simulink model "Template_v5_0_0_2026a_Original"  (R2026a)
settings: Solver=ode4  StopTime=tsim  FixedStep=baseRate  RelTol=1e-6  AbsTol=1e-6
undefined symbols (not defined in the file or in its folder): baseRate, dataRate, DiscIntNeverNeededParam, F_thrusters_BLACK, F_thrusters_BLUE, F_thrusters_RED, home_states_BLACK, home_states_BLUE, home_states_RED, IBLACK, IBLUE, init_states_BLACK, init_states_BLUE, init_states_RED, IRED, K_BLACK, K_BLUE, K_RED, labConsoleIP, mBLACK, mBLUE, mRED, Phase0_End, Phase1_End, Phase2_End, Phase3_End, Phase3_SubPhase1_End, Phase3_SubPhase2_End, Phase3_SubPhase3_End, Phase3_SubPhase4_End, Phase4_End, Phase5_End, platformSelection, PWMFreq, serverRate, simMode, tableDamping_BLACK, tableDamping_BLUE, tableDamping_RED, tableSlope, thrust_decay_BLACK, thrust_decay_BLUE, thrust_decay_RED, thruster_dist2CG_BLACK, thruster_dist2CG_BLUE, thruster_dist2CG_RED, xLength, yLength
libraries: simulink x18, dspinverses x3, nvidiaCommlib x1
(part 4 of 7)

== system Template_v5_0_0_2026a_Original/PhaseSpace Camera Code/Use Hardware to Obtain States/Store RED Data ==
  note: Store RED Position and Velocity Data
  RED Data : Inport
  RED Velocities : Inport  Port=2
  PS Clock : Inport  Port=3
  Calculate True Time Step : Subsystem
      settings: PortSchema="{\"entries\":[{\"content\":{\"sides\":[{\"content\":{\"connectorIds\":[\"In1\"]},\"type\":\"ConnectorPlacement.EquallySpacedRectSide\",\"uuid\":\"62932c5c-f2a7-44c8-96b4-4a75bab3a126\"},{\"content\":{\"connectorIds\":[\"Out1\"],\"side\":\"RIGHT\"},\"type\":\"ConnectorPlacement.EquallySpacedRectSide\",\"uuid\":\"82b3b717-2171-4047-b0df-3cd41cf9dfc7\"},{\"content\":{\"side\":\"TOP\"},\"type\":\"ConnectorPlacement.EquallySpacedRectSide\",\"uuid\":\"a142272a-a0ff-4882-8a2d-4633b3c7e02f\"},{\"content\":{\"connectorIds\":[\"In2\"],\"side\":\"BOTTOM\"},\"type\":\"ConnectorPlacement.EquallySpacedRectSide\",\"uuid\":\"b1e1ff4c-66d6-488f-92fb-77f76780833b\"}]},\"type\":\"ConnectorPlacement.EquallySpacedConnector\",\"uuid\":\"98c51868-8a10-4b52-aae4-56f6042c65c4\"}],\"packageUris\":[\"http://schema.mathworks.com/mf0/Connector/R2020b\"],\"version\":\"1.0\"}"
  Convert REDVX from [mm] to [m] : Gain  Gain=1/1000
  Convert REDVY from [mm] to [m] : Gain  Gain=1/1000
  Convert REDX from [mm] to [m] : Gain  Gain=1/1000
  Convert REDY from [mm] to [m] : Gain  Gain=1/1000
  Demux : Demux  Outputs=3
  Demux1 : Demux
  Demux2 : Demux  Outputs=3
  Mux{1..4} (4 alike) : Mux  Inputs=3
  RED_Px7 : DataStoreWrite  DataStoreName=RED_Measured_States  IndexOptions=Index vector (dialog)  Indices=1  OutputSizes=1
  Reshape : Reshape  OutputDimensionality=Column vector (2-D)
  Subsystem1 : Subsystem
  Subsystem2 : Subsystem
  Universal_Time : DataStoreWrite  DataStoreName=Univ_Time  IndexOptions=Index vector (dialog)  Indices=1  OutputSizes=1
  Wrap : Subsystem
  wires:
  Demux1/2 -> Convert REDX from [mm] to [m]/1
  Demux1/3 -> Convert REDY from [mm] to [m]/1
  RED Data/1 -> Demux1/1
  Demux1/4 -> Mux3/3
  Demux1/1 -> Universal_Time/1
  Mux2/1 -> RED_Px7/1
  Reshape/1 -> Subsystem1/2(y)
  Wrap/1(Wrapped Angle) -> Mux1/3
  Demux/3 -> Wrap/1(Unwrapped Angle)
  Demux/1 -> Mux1/1
  Subsystem2/1(dy/dt) -> Reshape/1
  Mux3/1 -> Subsystem2/2(y), Demux/1, Calculate True Time Step/2(Data)
  Demux/2 -> Mux1/2
  Convert REDX from [mm] to [m]/1 -> Mux3/1
  Convert REDY from [mm] to [m]/1 -> Mux3/2
  Calculate True Time Step/1(dt_out) -> Subsystem2/1(dt), Subsystem1/1(dt)
  Mux1/1 -> Mux2/1
  Subsystem1/1(dy/dt) -> Mux2/3
  Convert REDVX from [mm] to [m]/1 -> Mux4/1
  Convert REDVY from [mm] to [m]/1 -> Mux4/2
  Demux2/1 -> Convert REDVX from [mm] to [m]/1
  Demux2/2 -> Convert REDVY from [mm] to [m]/1
  Demux2/3 -> Mux4/3
  RED Velocities/1 -> Demux2/1
  Mux4/1 -> Mux2/2
  PS Clock/1 -> Calculate True Time Step/1(Time)

== system Template_v5_0_0_2026a_Original/Simulate Plant Dynamics/BLACK Dynamics/Calculated & Store Measured States ==
  y : Inport
  dt : Inport  Port=2
  Demux : Demux  Outputs=3
  Measured States for BLACK : DataStoreWrite  DataStoreName=BLACK_Measured_States  IndexOptions=Index vector (dialog)  Indices=1  OutputSizes=1
  Mux1 : Mux  Inputs=3
  Mux2 : Mux  Inputs=3
  Reshape : Reshape  OutputDimensionality=Column vector (2-D)
  Subsystem1 : Subsystem
  Subsystem2 : Subsystem
  Wrap : Subsystem
  wires:
  Demux/1 -> Mux1/1
  Wrap/1(Wrapped Angle) -> Mux1/3
  Demux/3 -> Wrap/1(Unwrapped Angle)
  Demux/2 -> Mux1/2
  Mux2/1 -> Measured States for BLACK/1
  Reshape/1 -> Subsystem1/2(y)
  Subsystem2/1(dy/dt) -> Mux2/2, Reshape/1
  y/1 -> Subsystem2/2(y), Demux/1
  Mux1/1 -> Mux2/1
  Subsystem1/1(dy/dt) -> Mux2/3
  dt/1 -> Subsystem1/1(dt), Subsystem2/1(dt)

== system Template_v5_0_0_2026a_Original/Simulate Plant Dynamics/BLACK Dynamics/Calculated & Store True States ==
  y : Inport
  Demux : Demux  Outputs=3
  Discrete Derivative : simulink/Discrete/Discrete Derivative  gainval=1.0  ICPrevScaledInput=0.0  OutMin=[]  OutMax=[]  OutDataType=fixdt(1, 16)  OutScaling=2^-10  DoSatur=off
  Discrete Derivative1 : simulink/Discrete/Discrete Derivative  gainval=1.0  ICPrevScaledInput=0.0  OutMin=[]  OutMax=[]  OutDataType=fixdt(1, 16)  OutScaling=2^-10  DoSatur=off
  Mux1 : Mux  Inputs=3
  Mux2 : Mux  Inputs=3
  True States for BLACK : DataStoreWrite  DataStoreName=BLACK_True_States  IndexOptions=Index vector (dialog)  Indices=1  OutputSizes=1
  Wrap : Subsystem
  wires:
  Demux/1 -> Mux1/1
  Wrap/1(Wrapped Angle) -> Mux1/3
  Demux/3 -> Wrap/1(Unwrapped Angle)
  Demux/2 -> Mux1/2
  Mux2/1 -> True States for BLACK/1
  y/1 -> Discrete Derivative/1, Demux/1
  Discrete Derivative/1 -> Mux2/2, Discrete Derivative1/1
  Mux1/1 -> Mux2/1
  Discrete Derivative1/1 -> Mux2/3

== system Template_v5_0_0_2026a_Original/Simulate Plant Dynamics/BLACK Dynamics/Data @ Measurement Rate ==
  Data Input : Inport
  Calculate True Time Step : Subsystem
  Constant1 : Constant  Value=dataRate
  Constant2 : Constant  Value=0
  Data Store Read : DataStoreRead  DataStoreName=Univ_Time  IndexOptions=Index vector (dialog)  Indices=1  OutputSizes=1
  Delay : Delay  DelayLength=1
  Enabled Subsystem : Subsystem  TreatAsAtomicUnit=on
  Enabled Subsystem1 : Subsystem  TreatAsAtomicUnit=on
  Relational Operator1 : RelationalOperator  OutDataTypeStr=boolean  RndMeth=Simplest  InputSameDT=off
  Relational Operator2 : RelationalOperator  Operator===  OutDataTypeStr=boolean  RndMeth=Simplest  InputSameDT=off
  Subtract : Sum  Inputs=+-
  Data Held : Outport
  Time Step : Outport  Port=2
  wires:
  Data Input/1 -> Enabled Subsystem1/1(ThrustPer_Final)
  Subtract/1 -> Relational Operator2/1, Delay/1
  Relational Operator2/1 -> Enabled Subsystem1/Enable
  Relational Operator1/1 -> Enabled Subsystem/Enable
  Constant1/1 -> Calculate True Time Step/3(Rate), Relational Operator1/2
  Constant2/1 -> Relational Operator2/2
  Enabled Subsystem/1(Out1) -> Calculate True Time Step/2(Time), Subtract/2
  Delay/1 -> Relational Operator1/1
  Data Store Read/1 -> Enabled Subsystem/1(In1), Subtract/1
  Enabled Subsystem1/1(Out1) -> Calculate True Time Step/1(Data), Data Held/1
  Calculate True Time Step/1(dt_out) -> Time Step/1

== system Template_v5_0_0_2026a_Original/Simulate Plant Dynamics/BLACK Dynamics/Dynamics Model for BLACK ==
  control_inputs : Inport
  Acceleration to Velocity : DiscreteIntegrator  IntegratorMethod=Integration: Backward Euler  SampleTime=-1  ICPrevOutput=DiscIntNeverNeededParam  ICPrevScaledInput=DiscIntNeverNeededParam
  Float State : DataStoreRead  DataStoreName=Float_State  IndexOptions=Index vector (dialog)  Indices=1  OutputSizes=1
  MATLAB Function : MATLAB Function  TreatAsAtomicUnit=on
  Previous Position : UnitDelay  InitialCondition=init_states_BLACK(:)  SampleTime=-1
  Previous Velocity : UnitDelay  InitialCondition=[0; 0; 0]  SampleTime=-1
  Velocity to Position : DiscreteIntegrator  IntegratorMethod=Integration: Backward Euler  InitialCondition=init_states_BLACK  SampleTime=-1  ICPrevOutput=DiscIntNeverNeededParam  ICPrevScaledInput=DiscIntNeverNeededParam
  states : Outport  VectorParamsAs1DForOutWhenUnconnected=off
  wires:
  control_inputs/1 -> MATLAB Function/1(control_inputs)
  MATLAB Function/1(x_ddot) -> Acceleration to Velocity/1
  Acceleration to Velocity/1 -> Velocity to Position/1, Previous Velocity/1
  Velocity to Position/1 -> states/1, Previous Position/1
  Previous Position/1 -> MATLAB Function/2(position)
  Previous Velocity/1 -> MATLAB Function/3(velocity)
  Float State/1 -> MATLAB Function/4(floating)

== system Template_v5_0_0_2026a_Original/Simulate Plant Dynamics/BLUE Dynamics/BLUE  Dynamics Model ==
  control_inputs : Inport
  Acceleration to Velocity : DiscreteIntegrator  IntegratorMethod=Integration: Backward Euler  SampleTime=-1  ICPrevOutput=DiscIntNeverNeededParam  ICPrevScaledInput=DiscIntNeverNeededParam
  Float State : DataStoreRead  DataStoreName=Float_State  IndexOptions=Index vector (dialog)  Indices=1  OutputSizes=1
  MATLAB Function : MATLAB Function  TreatAsAtomicUnit=on
  Previous Position : UnitDelay  InitialCondition=init_states_BLUE(:)  SampleTime=-1
  Previous Velocity : UnitDelay  InitialCondition=[0; 0; 0]  SampleTime=-1
  Velocity to Position : DiscreteIntegrator  IntegratorMethod=Integration: Backward Euler  InitialCondition=init_states_BLUE  SampleTime=-1  ICPrevOutput=DiscIntNeverNeededParam  ICPrevScaledInput=DiscIntNeverNeededParam
  states : Outport  VectorParamsAs1DForOutWhenUnconnected=off
  wires:
  control_inputs/1 -> MATLAB Function/1(control_inputs)
  MATLAB Function/1(x_ddot) -> Acceleration to Velocity/1
  Acceleration to Velocity/1 -> Velocity to Position/1, Previous Velocity/1
  Velocity to Position/1 -> states/1, Previous Position/1
  Previous Position/1 -> MATLAB Function/2(position)
  Previous Velocity/1 -> MATLAB Function/3(velocity)
  Float State/1 -> MATLAB Function/4(floating)

== system Template_v5_0_0_2026a_Original/Simulate Plant Dynamics/BLUE Dynamics/Calculated & Store Measured States ==
  y : Inport
  dt : Inport  Port=2
  Demux : Demux  Outputs=3
  Measured States for BLUE : DataStoreWrite  DataStoreName=BLUE_Measured_States  IndexOptions=Index vector (dialog)  Indices=1  OutputSizes=1
  Mux1 : Mux  Inputs=3
  Mux2 : Mux  Inputs=3
  Reshape : Reshape  OutputDimensionality=Column vector (2-D)
  Subsystem1 : Subsystem
  Subsystem2 : Subsystem
  Wrap : Subsystem
  wires:
  Demux/1 -> Mux1/1
  Wrap/1(Wrapped Angle) -> Mux1/3
  Demux/3 -> Wrap/1(Unwrapped Angle)
  Demux/2 -> Mux1/2
  Mux2/1 -> Measured States for BLUE/1
  Reshape/1 -> Subsystem1/2(y)
  Subsystem2/1(dy/dt) -> Mux2/2, Reshape/1
  y/1 -> Subsystem2/2(y), Demux/1
  dt/1 -> Subsystem1/1(dt), Subsystem2/1(dt)
  Subsystem1/1(dy/dt) -> Mux2/3
  Mux1/1 -> Mux2/1

== system Template_v5_0_0_2026a_Original/Simulate Plant Dynamics/BLUE Dynamics/Calculated & Store True States ==
  y : Inport
  Demux : Demux  Outputs=3
  Discrete Derivative : simulink/Discrete/Discrete Derivative  gainval=1.0  ICPrevScaledInput=0.0  OutMin=[]  OutMax=[]  OutDataType=fixdt(1, 16)  OutScaling=2^-10  DoSatur=off
  Discrete Derivative1 : simulink/Discrete/Discrete Derivative  gainval=1.0  ICPrevScaledInput=0.0  OutMin=[]  OutMax=[]  OutDataType=fixdt(1, 16)  OutScaling=2^-10  DoSatur=off
  Mux1 : Mux  Inputs=3
  Mux2 : Mux  Inputs=3
  True States for BLUE : DataStoreWrite  DataStoreName=BLUE_True_States  IndexOptions=Index vector (dialog)  Indices=1  OutputSizes=1
  Wrap : Subsystem
  wires:
  Demux/1 -> Mux1/1
  Wrap/1(Wrapped Angle) -> Mux1/3
  Demux/3 -> Wrap/1(Unwrapped Angle)
  Demux/2 -> Mux1/2
  Mux2/1 -> True States for BLUE/1
  Mux1/1 -> Mux2/1
  y/1 -> Discrete Derivative/1, Demux/1
  Discrete Derivative/1 -> Discrete Derivative1/1, Mux2/2
  Discrete Derivative1/1 -> Mux2/3

== system Template_v5_0_0_2026a_Original/Simulate Plant Dynamics/BLUE Dynamics/Data @ Measurement Rate ==
  Data Input : Inport
  Calculate True Time Step : Subsystem
  Constant1 : Constant  Value=dataRate
  Constant2 : Constant  Value=0
  Data Store Read : DataStoreRead  DataStoreName=Univ_Time  IndexOptions=Index vector (dialog)  Indices=1  OutputSizes=1
  Delay : Delay  DelayLength=1
  Enabled Subsystem : Subsystem  TreatAsAtomicUnit=on
  Enabled Subsystem1 : Subsystem  TreatAsAtomicUnit=on
  Relational Operator1 : RelationalOperator  OutDataTypeStr=boolean  RndMeth=Simplest  InputSameDT=off
  Relational Operator2 : RelationalOperator  Operator===  OutDataTypeStr=boolean  RndMeth=Simplest  InputSameDT=off
  Subtract : Sum  Inputs=+-
  Data Held : Outport
  Time Step : Outport  Port=2
  wires:
  Data Input/1 -> Enabled Subsystem1/1(ThrustPer_Final)
  Subtract/1 -> Relational Operator2/1, Delay/1
  Relational Operator2/1 -> Enabled Subsystem1/Enable
  Relational Operator1/1 -> Enabled Subsystem/Enable
  Constant1/1 -> Calculate True Time Step/3(Rate), Relational Operator1/2
  Constant2/1 -> Relational Operator2/2
  Enabled Subsystem/1(Out1) -> Calculate True Time Step/2(Time), Subtract/2
  Delay/1 -> Relational Operator1/1
  Data Store Read/1 -> Enabled Subsystem/1(In1), Subtract/1
  Enabled Subsystem1/1(Out1) -> Calculate True Time Step/1(Data), Data Held/1
  Calculate True Time Step/1(dt_out) -> Time Step/1

== system Template_v5_0_0_2026a_Original/Simulate Plant Dynamics/RED and ARM Dynamics/RED + ARM ==
  note: RED + ARM Plant (spot.arm.Plant): the base, the arm and its three Dynamixel servos in PWM control, with their back-EMF and friction, integrated at armModel.innerStep (1 ms) within each diagram step. Its arm input is what the real servos get: ARM_Controls, each joint's PWM [885 = 100 %]; it writes ARM_Measured_PWM, the PWM each servo applies. Parameters: armModel (spot.arm.parameters; friction and back-EMF from the project's arm calibration when there is one).
  Action Port : ActionPort  ActionPortLabel=if(u1 == 4 | u1 == 5 | u1 == 10 | u1 == 11)
  Add Noise : RandomNumber  Variance=1e-9  SampleTime=baseRate
  Calculated & Store Measured States : Subsystem
  Calculated & Store True States : Subsystem
  Data @ Measurement Rate : Subsystem
  Data Store Read3 : DataStoreRead  DataStoreName=ARM_Controls  IndexOptions=Index vector (dialog)  Indices=1  OutputSizes=1
  Data Store Write : DataStoreWrite  DataStoreName=ARM_Measured_States  IndexOptions=Index vector (dialog)  Indices=1  OutputSizes=1
  Data Store Write1 : DataStoreWrite  DataStoreName=ARM_Measured_PWM  IndexOptions=Index vector (dialog)  Indices=1  OutputSizes=1
  Demux : Demux  Outputs=[1,1,10]
  Encoder Pulses : Quantizer  QuantizationInterval=2*pi/4096
  Exceeded Table Limits : Subsystem
  Float State : DataStoreRead  DataStoreName=Float_State  IndexOptions=Index vector (dialog)  Indices=1  OutputSizes=1
  Joint Angles : Selector  InputPortWidth=6  IndexOptions=Index vector (dialog)  Indices=[4 5 6]  OutputSizes=1
  Joint Rates : Selector  InputPortWidth=6  IndexOptions=Index vector (dialog)  Indices=[4 5 6]  OutputSizes=1
  Mux : Mux  Inputs=2
  Mux Encoders : Mux  Inputs=2
  RED + ARM Plant : MATLABSystem  System=spot.arm.Plant  Model=armModel  FixedBase=off  FloatInput=on  SimulateUsing=Code generation
      mask Type: spot.arm.Plant
  Saturated Control Commands for RED : DataStoreRead  DataStoreName=RED_Saturated_Controls  IndexOptions=Index vector (dialog)  Indices=1  OutputSizes=1
  Stop Simulation : Stop
  Sum : Sum  Inputs=++|
  Terminator : Terminator
  Velocity Units : Quantizer  QuantizationInterval=0.229*2*pi/60
  wires:
  Data @ Measurement Rate/2(Time Step) -> Calculated & Store Measured States/2(dt)
  Mux/1 -> Demux/1
  Demux/1 -> Exceeded Table Limits/1(X)
  Exceeded Table Limits/1(Stop) -> Stop Simulation/1
  Demux/2 -> Exceeded Table Limits/2(Y)
  Demux/3 -> Terminator/1
  Add Noise/1 -> Sum/1
  Sum/1 -> Data @ Measurement Rate/1(Data Input)
  Data @ Measurement Rate/1(Data Held) -> Calculated & Store Measured States/1(y)
  Saturated Control Commands for RED/1 -> RED + ARM Plant/1
  RED + ARM Plant/1 -> Calculated & Store True States/1(y), Sum/2, Mux/1, Joint Angles/1
  RED + ARM Plant/2 -> Mux/2, Joint Rates/1
  Data Store Read3/1 -> RED + ARM Plant/2
  Joint Angles/1 -> Encoder Pulses/1
  Joint Rates/1 -> Velocity Units/1
  Encoder Pulses/1 -> Mux Encoders/1
  Velocity Units/1 -> Mux Encoders/2
  Mux Encoders/1 -> Data Store Write/1
  RED + ARM Plant/3 -> Data Store Write1/1
  Float State/1 -> RED + ARM Plant/3

== system Template_v5_0_0_2026a_Original/Simulate Plant Dynamics/RED and ARM Dynamics/RED Only ==
  Action Port : ActionPort  ActionPortLabel=else
  Add Noise : RandomNumber  Variance=1e-9  SampleTime=baseRate
  Calculated & Store Measured States : Subsystem
  Calculated & Store True States : Subsystem
  Data @ Measurement Rate : Subsystem
  Dynamics Model for RED : Subsystem  SystemSampleTime=serverRate
      settings: PortSchema="{\"entries\":[{\"content\":{\"sides\":[{\"content\":{\"connectorIds\":[\"In1\"]},\"type\":\"ConnectorPlacement.EquallySpacedRectSide\",\"uuid\":\"36f8472d-4371-4b5e-bb25-792dc7798e2d\"},{\"content\":{\"side\":\"RIGHT\"},\"type\":\"ConnectorPlacement.EquallySpacedRectSide\",\"uuid\":\"cd500640-3349-40a3-88e5-d39ca64affda\"},{\"content\":{\"connectorIds\":[\"Out1\"],\"side\":\"TOP\"},\"type\":\"ConnectorPlacement.EquallySpacedRectSide\",\"uuid\":\"f35070a8-6b00-4762-8673-30fcbcb2fe63\"}]},\"type\":\"ConnectorPlacement.EquallySpacedConnector\",\"uuid\":\"7478ab5e-be27-4ef2-a158-875ec93c8619\"}],\"packageUris\":[\"http://schema.mathworks.com/mf0/Connector/R2020b\"],\"version\":\"1.0\"}"
  Saturated Control Commands for RED : DataStoreRead  DataStoreName=RED_Saturated_Controls  IndexOptions=Index vector (dialog)  Indices=1  OutputSizes=1
  Sum : Sum  Inputs=++|
  wires:
  Saturated Control Commands for RED/1 -> Dynamics Model for RED/1(control_inputs)
  Data @ Measurement Rate/2(Time Step) -> Calculated & Store Measured States/2(dt)
  Data @ Measurement Rate/1(Data Held) -> Calculated & Store Measured States/1(y)
  Add Noise/1 -> Sum/1
  Dynamics Model for RED/1(states) -> Sum/2, Calculated & Store True States/1(y)
  Sum/1 -> Data @ Measurement Rate/1(Data Input)

== system Template_v5_0_0_2026a_Original/Thruster & Float Control Code/Change BLACK Behavior/Calculate Duty Cycle ==
  "[Fx_b; Fy_b; Tz]" : Inport
  Measured Attitude : Inport  Port=2
  Demux : Demux  Outputs=3
  Duty Cycle @ PWM : Subsystem
  Generate Initial Guess : Subsystem
  MATLAB Function1 : MATLAB Function  TreatAsAtomicUnit=on
  MATLAB Function5 : MATLAB Function  TreatAsAtomicUnit=on  mask{max_iters=20, tol=1e-6}
      mask prompts: max_iters "Maximum Number of Iterations"; tol "Convergence Tolerance"
  Mux : Mux  Inputs=2
  Mux1 : Mux  Inputs=2
  Product1 : Product  Multiplication=Matrix(*)
  Reshape : Reshape  OutputDimensionality=Column vector (2-D)
  Rotate Forces to Inertial : Subsystem
  Duty Cycle : Outport  VectorParamsAs1DForOutWhenUnconnected=off
  Saturated Forces Moments : Outport  Port=2
  wires:
  Rotate Forces to Inertial/1(F_I) -> Mux1/1
  Generate Initial Guess/1(Duty Cycle) -> MATLAB Function5/2(x0)
  Product1/1 -> Demux/1
  Measured Attitude/1 -> Rotate Forces to Inertial/2(Rz)
  Duty Cycle @ PWM/1(Duty Cycle Held) -> Product1/2
  "[Fx_b; Fy_b; Tz]"/1 -> Generate Initial Guess/1("[Fx; Fy; Tz]"), Reshape/1
  MATLAB Function5/2(duty_cycles) -> MATLAB Function1/1(ThrustPer), Duty Cycle/1
  Demux/2 -> Mux/2
  Mux/1 -> Rotate Forces to Inertial/1("F_b ")
  Demux/3 -> Mux1/2
  Demux/1 -> Mux/1
  Reshape/1 -> MATLAB Function5/1(u_desired)
  MATLAB Function5/1(H_final) -> Product1/1
  Mux1/1 -> Saturated Forces Moments/1
  MATLAB Function1/1(ThrustPer_Final) -> Duty Cycle @ PWM/1(ThrustPer_Final)

== system Template_v5_0_0_2026a_Original/Thruster & Float Control Code/Change BLACK Behavior/Rotate Forces to Body ==
  "F_I " : Inport
  Rz : Inport  Port=2
  Create Rotation Matrix : MATLAB Function  TreatAsAtomicUnit=on
  Rotate F_I to F_b : Product  Multiplication=Matrix(*)
  F_b : Outport  VectorParamsAs1DForOutWhenUnconnected=off
  wires:
  Rotate F_I to F_b/1 -> F_b/1
  Create Rotation Matrix/1(C_bI) -> Rotate F_I to F_b/1
  "F_I "/1 -> Rotate F_I to F_b/2
  Rz/1 -> Create Rotation Matrix/1(Rz)

== system Template_v5_0_0_2026a_Original/Thruster & Float Control Code/Change BLUE Behavior/Calculate Duty Cycle ==
  "[Fx_b; Fy_b; Tz]" : Inport
  Measured Attitude : Inport  Port=2
  Demux : Demux  Outputs=3
  Duty Cycle @ PWM : Subsystem
  Generate Initial Guess : Subsystem
  MATLAB Function1 : MATLAB Function  TreatAsAtomicUnit=on
  MATLAB Function5 : MATLAB Function  TreatAsAtomicUnit=on  mask{max_iters=20, tol=1e-6}
      mask prompts: max_iters "Maximum Number of Iterations"; tol "Convergence Tolerance"
  Mux : Mux  Inputs=2
  Mux1 : Mux  Inputs=2
  Product1 : Product  Multiplication=Matrix(*)
  Reshape : Reshape  OutputDimensionality=Column vector (2-D)
  Rotate Forces to Inertial : Subsystem
  Duty Cycle : Outport  VectorParamsAs1DForOutWhenUnconnected=off
  Saturated Forces Moments : Outport  Port=2
  wires:
  Rotate Forces to Inertial/1(F_I) -> Mux1/1
  Generate Initial Guess/1(Duty Cycle) -> MATLAB Function5/2(x0)
  Product1/1 -> Demux/1
  Measured Attitude/1 -> Rotate Forces to Inertial/2(Rz)
  Duty Cycle @ PWM/1(Duty Cycle Held) -> Product1/2
  "[Fx_b; Fy_b; Tz]"/1 -> Generate Initial Guess/1("[Fx; Fy; Tz]"), Reshape/1
  MATLAB Function5/2(duty_cycles) -> Duty Cycle/1, MATLAB Function1/1(ThrustPer)
  Demux/2 -> Mux/2
  Mux/1 -> Rotate Forces to Inertial/1("F_b ")
  Demux/3 -> Mux1/2
  Demux/1 -> Mux/1
  Reshape/1 -> MATLAB Function5/1(u_desired)
  Mux1/1 -> Saturated Forces Moments/1
  MATLAB Function5/1(H_final) -> Product1/1
  MATLAB Function1/1(ThrustPer_Final) -> Duty Cycle @ PWM/1(ThrustPer_Final)

== system Template_v5_0_0_2026a_Original/Thruster & Float Control Code/Change BLUE Behavior/Rotate Forces to Body ==
  "F_I " : Inport
  Rz : Inport  Port=2
  Create Rotation Matrix : MATLAB Function  TreatAsAtomicUnit=on
  Rotate F_I to F_b : Product  Multiplication=Matrix(*)
  F_b : Outport  VectorParamsAs1DForOutWhenUnconnected=off
  wires:
  Rotate F_I to F_b/1 -> F_b/1
  Create Rotation Matrix/1(C_bI) -> Rotate F_I to F_b/1
  "F_I "/1 -> Rotate F_I to F_b/2
  Rz/1 -> Create Rotation Matrix/1(Rz)

== system Template_v5_0_0_2026a_Original/Thruster & Float Control Code/Change RED Behavior/Calculate Duty Cycle ==
  "[Fx_b; Fy_b; Tz]" : Inport
  Measured Attitude : Inport  Port=2
  Demux : Demux  Outputs=3
  Duty Cycle @ PWM : Subsystem
  Generate Initial Guess : Subsystem
  MATLAB Function5 : MATLAB Function  TreatAsAtomicUnit=on  mask{max_iters=20, tol=1e-6}
      mask prompts: max_iters "Maximum Number of Iterations"; tol "Convergence Tolerance"
  MATLAB Function8 : MATLAB Function  TreatAsAtomicUnit=on
  Mux : Mux  Inputs=2
  Mux1 : Mux  Inputs=2
  Product1 : Product  Multiplication=Matrix(*)
  Reshape : Reshape  OutputDimensionality=Column vector (2-D)
  Rotate Forces to Inertial : Subsystem
  Duty Cycle : Outport  VectorParamsAs1DForOutWhenUnconnected=off
  Saturated Forces Moments : Outport  Port=2
  wires:
  Demux/2 -> Mux/2
  Measured Attitude/1 -> Rotate Forces to Inertial/2(Rz)
  Rotate Forces to Inertial/1(F_I) -> Mux1/1
  Product1/1 -> Demux/1
  Demux/1 -> Mux/1
  Mux/1 -> Rotate Forces to Inertial/1("F_b ")
  Demux/3 -> Mux1/2
  Reshape/1 -> MATLAB Function5/1(u_desired)
  MATLAB Function5/1(H_final) -> Product1/1
  MATLAB Function5/2(duty_cycles) -> Duty Cycle/1, MATLAB Function8/1(ThrustPer)
  Duty Cycle @ PWM/1(Duty Cycle Held) -> Product1/2
  Generate Initial Guess/1(Duty Cycle) -> MATLAB Function5/2(x0)
  Mux1/1 -> Saturated Forces Moments/1
  MATLAB Function8/1(ThrustPer_Final) -> Duty Cycle @ PWM/1(ThrustPer_Final)
  "[Fx_b; Fy_b; Tz]"/1 -> Reshape/1, Generate Initial Guess/1("[Fx; Fy; Tz]")

== system Template_v5_0_0_2026a_Original/Thruster & Float Control Code/Change RED Behavior/Rotate Forces to Body ==
  "F_I " : Inport
  Rz : Inport  Port=2
  Create Rotation Matrix : MATLAB Function  TreatAsAtomicUnit=on
  Rotate F_I to F_b : Product  Multiplication=Matrix(*)
  F_b : Outport  VectorParamsAs1DForOutWhenUnconnected=off
  wires:
  Rotate F_I to F_b/1 -> F_b/1
  Create Rotation Matrix/1(C_bI) -> Rotate F_I to F_b/1
  "F_I "/1 -> Rotate F_I to F_b/2
  Rz/1 -> Create Rotation Matrix/1(Rz)

== system Template_v5_0_0_2026a_Original/1 - Experiment Logic/Phase #3: Experiment/Sub-Phase #1/Desired Joint Angles RED ==
  Constant1 : Constant  Value=pi/2
  Constant2 : Constant  Value=0
  Constant3 : Constant  Value=0
  Mux : Mux  Inputs=3
  Target Array : Outport
  wires:
  Mux/1 -> Target Array/1
  Constant3/1 -> Mux/1
  Constant1/1 -> Mux/2
  Constant2/1 -> Mux/3

== system Template_v5_0_0_2026a_Original/1 - Experiment Logic/Phase #3: Experiment/Sub-Phase #1/Desired Position BLACK ==
  Calculate Circular Tracking : Subsystem
  Calculate Time since Phase #3 Start : Subsystem
  Constant : Constant  Value=2*pi/3
  "Desired Rate " : Constant  Value=0.03490659  SampleTime=-1
  Mux : Mux  Inputs=3
  Product : Product
  Sum : Sum  Inputs=|++
  Wrap : Subsystem
  Target Array : Outport
  wires:
  Mux/1 -> Target Array/1
  Calculate Time since Phase #3 Start/1(Time) -> Product/2
  Constant/1 -> Calculate Circular Tracking/2(Phase), Sum/2
  "Desired Rate "/1 -> Product/1
  Product/1 -> Calculate Circular Tracking/1(Angular Frequency), Sum/1
  Sum/1 -> Wrap/1(In1)
  Wrap/1(Out1) -> Mux/3
  Calculate Circular Tracking/1(Target X) -> Mux/1
  Calculate Circular Tracking/2(Target Y) -> Mux/2

== system Template_v5_0_0_2026a_Original/1 - Experiment Logic/Phase #3: Experiment/Sub-Phase #1/Desired Position BLUE ==
  Calculate Circular Tracking : Subsystem
  Calculate Time since Phase #3 Start : Subsystem
  Constant : Constant  Value=4*pi/3
  "Desired Rate " : Constant  Value=0.03490659  SampleTime=-1
  Mux : Mux  Inputs=3
  Product : Product
  Sum : Sum  Inputs=|++
  Wrap : Subsystem
  Target Array : Outport
  wires:
  Mux/1 -> Target Array/1
  Calculate Time since Phase #3 Start/1(Time) -> Product/2
  Constant/1 -> Calculate Circular Tracking/2(Phase), Sum/2
  "Desired Rate "/1 -> Product/1
  Product/1 -> Calculate Circular Tracking/1(Angular Frequency), Sum/1
  Sum/1 -> Wrap/1(In1)
  Wrap/1(Out1) -> Mux/3
  Calculate Circular Tracking/1(Target X) -> Mux/1
  Calculate Circular Tracking/2(Target Y) -> Mux/2

== system Template_v5_0_0_2026a_Original/1 - Experiment Logic/Phase #3: Experiment/Sub-Phase #1/Desired Position RED ==
  Calculate Circular Tracking : Subsystem
  Calculate Time since Phase #3 Start : Subsystem
  Constant : Constant  Value=0
  "Desired Rate " : Constant  Value=0.03490659  SampleTime=-1
  Mux : Mux  Inputs=3
  Product : Product
  Sum : Sum  Inputs=|++
  Wrap : Subsystem
  Target Array : Outport
  wires:
  Mux/1 -> Target Array/1
  Calculate Time since Phase #3 Start/1(Time) -> Product/2
  Constant/1 -> Calculate Circular Tracking/2(Phase), Sum/2
  "Desired Rate "/1 -> Product/1
  Product/1 -> Calculate Circular Tracking/1(Angular Frequency), Sum/1
  Sum/1 -> Wrap/1(In1)
  Wrap/1(Out1) -> Mux/3
  Calculate Circular Tracking/1(Target X) -> Mux/1
  Calculate Circular Tracking/2(Target Y) -> Mux/2

== system Template_v5_0_0_2026a_Original/1 - Experiment Logic/Phase #3: Experiment/Sub-Phase #2/Desired Joint Angles RED ==
  Constant1 : Constant  Value=pi/2
  Constant2 : Constant  Value=0
  Constant3 : Constant  Value=pi/2
  Mux : Mux  Inputs=3
  Target Array : Outport
  wires:
  Mux/1 -> Target Array/1
  Constant3/1 -> Mux/1
  Constant1/1 -> Mux/2
  Constant2/1 -> Mux/3

== system Template_v5_0_0_2026a_Original/1 - Experiment Logic/Phase #3: Experiment/Sub-Phase #2/Desired Position BLACK ==
  Calculate Circular Tracking : Subsystem
  Calculate Time since Phase #3 Start : Subsystem
  Constant : Constant  Value=2*pi/3
  "Desired Rate " : Constant  Value=0.03490659  SampleTime=-1
  Mux : Mux  Inputs=3
  Product : Product
  Sum : Sum  Inputs=|++
  Wrap : Subsystem
  Target Array : Outport
  wires:
  Mux/1 -> Target Array/1
  Calculate Time since Phase #3 Start/1(Time) -> Product/2
  Constant/1 -> Calculate Circular Tracking/2(Phase), Sum/2
  "Desired Rate "/1 -> Product/1
  Product/1 -> Calculate Circular Tracking/1(Angular Frequency), Sum/1
  Sum/1 -> Wrap/1(In1)
  Wrap/1(Out1) -> Mux/3
  Calculate Circular Tracking/1(Target X) -> Mux/1
  Calculate Circular Tracking/2(Target Y) -> Mux/2

== system Template_v5_0_0_2026a_Original/1 - Experiment Logic/Phase #3: Experiment/Sub-Phase #2/Desired Position BLUE ==
  Calculate Circular Tracking : Subsystem
  Calculate Time since Phase #3 Start : Subsystem
  Constant : Constant  Value=4*pi/3
  "Desired Rate " : Constant  Value=0.03490659  SampleTime=-1
  Mux : Mux  Inputs=3
  Product : Product
  Sum : Sum  Inputs=|++
  Wrap : Subsystem
  Target Array : Outport
  wires:
  Mux/1 -> Target Array/1
  Calculate Time since Phase #3 Start/1(Time) -> Product/2
  Constant/1 -> Calculate Circular Tracking/2(Phase), Sum/2
  "Desired Rate "/1 -> Product/1
  Product/1 -> Calculate Circular Tracking/1(Angular Frequency), Sum/1
  Sum/1 -> Wrap/1(In1)
  Wrap/1(Out1) -> Mux/3
  Calculate Circular Tracking/1(Target X) -> Mux/1
  Calculate Circular Tracking/2(Target Y) -> Mux/2

== system Template_v5_0_0_2026a_Original/1 - Experiment Logic/Phase #3: Experiment/Sub-Phase #2/Desired Position RED ==
  Calculate Circular Tracking : Subsystem
  Calculate Time since Phase #3 Start : Subsystem
  Constant : Constant  Value=0
  "Desired Rate " : Constant  Value=0.03490659  SampleTime=-1
  Mux : Mux  Inputs=3
  Product : Product
  Sum : Sum  Inputs=|++
  Wrap : Subsystem
  Target Array : Outport
  wires:
  Mux/1 -> Target Array/1
  Calculate Time since Phase #3 Start/1(Time) -> Product/2
  Constant/1 -> Calculate Circular Tracking/2(Phase), Sum/2
  "Desired Rate "/1 -> Product/1
  Product/1 -> Calculate Circular Tracking/1(Angular Frequency), Sum/1
  Sum/1 -> Wrap/1(In1)
  Wrap/1(Out1) -> Mux/3
  Calculate Circular Tracking/1(Target X) -> Mux/1
  Calculate Circular Tracking/2(Target Y) -> Mux/2

== system Template_v5_0_0_2026a_Original/1 - Experiment Logic/Phase #3: Experiment/Sub-Phase #3/Desired Joint Angles RED ==
  Constant1 : Constant  Value=pi/2
  Constant2 : Constant  Value=0
  Constant3 : Constant  Value=pi/2
  Mux : Mux  Inputs=3
  Target Array : Outport
  wires:
  Mux/1 -> Target Array/1
  Constant3/1 -> Mux/1
  Constant1/1 -> Mux/2
  Constant2/1 -> Mux/3

== system Template_v5_0_0_2026a_Original/1 - Experiment Logic/Phase #3: Experiment/Sub-Phase #3/Desired Position BLACK ==
  Calculate Circular Tracking : Subsystem
  Calculate Time since Phase #3 Start : Subsystem
  Constant : Constant  Value=2*pi/3
  "Desired Rate " : Constant  Value=0.03490659  SampleTime=-1
  Mux : Mux  Inputs=3
  Product : Product
  Sum : Sum  Inputs=|++
  Wrap : Subsystem
  Target Array : Outport
  wires:
  Mux/1 -> Target Array/1
  Calculate Time since Phase #3 Start/1(Time) -> Product/2
  Constant/1 -> Calculate Circular Tracking/2(Phase), Sum/2
  "Desired Rate "/1 -> Product/1
  Product/1 -> Calculate Circular Tracking/1(Angular Frequency), Sum/1
  Sum/1 -> Wrap/1(In1)
  Wrap/1(Out1) -> Mux/3
  Calculate Circular Tracking/1(Target X) -> Mux/1
  Calculate Circular Tracking/2(Target Y) -> Mux/2

== system Template_v5_0_0_2026a_Original/1 - Experiment Logic/Phase #3: Experiment/Sub-Phase #3/Desired Position BLUE ==
  Calculate Circular Tracking : Subsystem
  Calculate Time since Phase #3 Start : Subsystem
  Constant : Constant  Value=4*pi/3
  "Desired Rate " : Constant  Value=0.03490659  SampleTime=-1
  Mux : Mux  Inputs=3
  Product : Product
  Sum : Sum  Inputs=|++
  Wrap : Subsystem
  Target Array : Outport
  wires:
  Mux/1 -> Target Array/1
  Calculate Time since Phase #3 Start/1(Time) -> Product/2
  Constant/1 -> Calculate Circular Tracking/2(Phase), Sum/2
  "Desired Rate "/1 -> Product/1
  Product/1 -> Calculate Circular Tracking/1(Angular Frequency), Sum/1
  Sum/1 -> Wrap/1(In1)
  Wrap/1(Out1) -> Mux/3
  Calculate Circular Tracking/1(Target X) -> Mux/1
  Calculate Circular Tracking/2(Target Y) -> Mux/2

== system Template_v5_0_0_2026a_Original/1 - Experiment Logic/Phase #3: Experiment/Sub-Phase #3/Desired Position RED ==
  Calculate Circular Tracking : Subsystem
  Calculate Time since Phase #3 Start : Subsystem
  Constant : Constant  Value=0
  "Desired Rate " : Constant  Value=0.03490659  SampleTime=-1
  Mux : Mux  Inputs=3
  Product : Product
  Sum : Sum  Inputs=|++
  Wrap : Subsystem
  Target Array : Outport
  wires:
  Mux/1 -> Target Array/1
  Calculate Time since Phase #3 Start/1(Time) -> Product/2
  Constant/1 -> Calculate Circular Tracking/2(Phase), Sum/2
  "Desired Rate "/1 -> Product/1
  Product/1 -> Calculate Circular Tracking/1(Angular Frequency), Sum/1
  Sum/1 -> Wrap/1(In1)
  Wrap/1(Out1) -> Mux/3
  Calculate Circular Tracking/1(Target X) -> Mux/1
  Calculate Circular Tracking/2(Target Y) -> Mux/2

== system Template_v5_0_0_2026a_Original/1 - Experiment Logic/Phase #3: Experiment/Sub-Phase #4/Desired Joint Angles RED ==
  Constant1 : Constant  Value=pi/2
  Constant2 : Constant  Value=0
  Constant3 : Constant  Value=pi/2
  Mux : Mux  Inputs=3
  Target Array : Outport
  wires:
  Mux/1 -> Target Array/1
  Constant3/1 -> Mux/1
  Constant1/1 -> Mux/2
  Constant2/1 -> Mux/3

== system Template_v5_0_0_2026a_Original/1 - Experiment Logic/Phase #3: Experiment/Sub-Phase #4/Desired Position BLACK ==
  Calculate Circular Tracking : Subsystem
  Calculate Time since Phase #3 Start : Subsystem
  Constant : Constant  Value=2*pi/3
  "Desired Rate " : Constant  Value=0.03490659  SampleTime=-1
  Mux : Mux  Inputs=3
  Product : Product
  Sum : Sum  Inputs=|++
  Wrap : Subsystem
  Target Array : Outport
  wires:
  Mux/1 -> Target Array/1
  Calculate Time since Phase #3 Start/1(Time) -> Product/2
  Constant/1 -> Calculate Circular Tracking/2(Phase), Sum/2
  "Desired Rate "/1 -> Product/1
  Product/1 -> Calculate Circular Tracking/1(Angular Frequency), Sum/1
  Sum/1 -> Wrap/1(In1)
  Wrap/1(Out1) -> Mux/3
  Calculate Circular Tracking/1(Target X) -> Mux/1
  Calculate Circular Tracking/2(Target Y) -> Mux/2

== system Template_v5_0_0_2026a_Original/1 - Experiment Logic/Phase #3: Experiment/Sub-Phase #4/Desired Position BLUE ==
  Calculate Circular Tracking : Subsystem
  Calculate Time since Phase #3 Start : Subsystem
  Constant : Constant  Value=4*pi/3
  "Desired Rate " : Constant  Value=0.03490659  SampleTime=-1
  Mux : Mux  Inputs=3
  Product : Product
  Sum : Sum  Inputs=|++
  Wrap : Subsystem
  Target Array : Outport
  wires:
  Mux/1 -> Target Array/1
  Calculate Time since Phase #3 Start/1(Time) -> Product/2
  Constant/1 -> Calculate Circular Tracking/2(Phase), Sum/2
  "Desired Rate "/1 -> Product/1
  Product/1 -> Calculate Circular Tracking/1(Angular Frequency), Sum/1
  Sum/1 -> Wrap/1(In1)
  Wrap/1(Out1) -> Mux/3
  Calculate Circular Tracking/1(Target X) -> Mux/1
  Calculate Circular Tracking/2(Target Y) -> Mux/2

== system Template_v5_0_0_2026a_Original/1 - Experiment Logic/Phase #3: Experiment/Sub-Phase #4/Desired Position RED ==
  Calculate Circular Tracking : Subsystem
  Calculate Time since Phase #3 Start : Subsystem
  Constant : Constant  Value=0
  "Desired Rate " : Constant  Value=0.03490659  SampleTime=-1
  Mux : Mux  Inputs=3
  Product : Product
  Sum : Sum  Inputs=|++
  Wrap : Subsystem
  Target Array : Outport
  wires:
  Mux/1 -> Target Array/1
  Calculate Time since Phase #3 Start/1(Time) -> Product/2
  Constant/1 -> Calculate Circular Tracking/2(Phase), Sum/2
  "Desired Rate "/1 -> Product/1
  Product/1 -> Calculate Circular Tracking/1(Angular Frequency), Sum/1
  Sum/1 -> Wrap/1(In1)
  Wrap/1(Out1) -> Mux/3
  Calculate Circular Tracking/1(Target X) -> Mux/1
  Calculate Circular Tracking/2(Target Y) -> Mux/2

== system Template_v5_0_0_2026a_Original/PhaseSpace Camera Code/Use Hardware to Obtain States/Receive and Process Phasespace Data/Experiment Clock ==
  packet : Inport
  age : Inport  Port=2
  Experiment Time : MATLAB Function  TreatAsAtomicUnit=on
  Send Sync. Time : Subsystem
  state : Terminator
  ClockAdjusted : Outport
  wires:
  packet/1 -> Experiment Time/1(packet)
  age/1 -> Experiment Time/2(age)
  Experiment Time/1(t) -> ClockAdjusted/1, Send Sync. Time/1(Universal Time)
  Experiment Time/2(state) -> state/1

== system Template_v5_0_0_2026a_Original/PhaseSpace Camera Code/Use Hardware to Obtain States/Store BLACK Data/Calculate True Time Step ==
  Time : Inport
  Data : Inport  Port=2
  Constant : Constant  Value=dataRate
  Constant3 : Constant  Value=0
  Delay1 : Delay  DelayLength=1  InitialCondition=0
  Delay2 : Delay  DelayLength=1  InitialCondition=0
  Demux : Demux  Outputs=3
  Enabled Subsystem3 : Subsystem  TreatAsAtomicUnit=on
  MATLAB Function : MATLAB Function  TreatAsAtomicUnit=on
  Relational Operator : RelationalOperator  Operator=~=  OutDataTypeStr=boolean  RndMeth=Simplest  InputSameDT=off
  Subtract1 : Sum  Inputs=+-
  Subtract2 : Sum  Inputs=+-
  Terminator : Terminator
  Terminator1 : Terminator
  dt_out : Outport
  wires:
  Demux/3 -> Terminator1/1
  Constant/1 -> MATLAB Function/2(dataRate)
  MATLAB Function/1(dt_out) -> dt_out/1
  Time/1 -> Delay2/1, Subtract1/1
  Enabled Subsystem3/1(dy(t)/dt) -> MATLAB Function/1(dt)
  Data/1 -> Demux/1
  Subtract2/1 -> Relational Operator/1
  Relational Operator/1 -> Enabled Subsystem3/Enable
  Constant3/1 -> Relational Operator/2
  Demux/1 -> Subtract2/1, Delay1/1
  Delay1/1 -> Subtract2/2
  Demux/2 -> Terminator/1
  Subtract1/1 -> Enabled Subsystem3/1(y2-y1)
  Delay2/1 -> Subtract1/2

== system Template_v5_0_0_2026a_Original/PhaseSpace Camera Code/Use Hardware to Obtain States/Store BLACK Data/Subsystem1 ==
  dt : Inport
  y : Inport  Port=2
  Constant3 : Constant  Value=0
  Delay1 : Delay  DelayLength=1
  Enabled Subsystem : Subsystem  TreatAsAtomicUnit=on
  Relational Operator : RelationalOperator  Operator=~=  OutDataTypeStr=boolean  RndMeth=Simplest  InputSameDT=off
  Subtract1 : Sum  Inputs=+-
  dy/dt : Outport
  wires:
  Constant3/1 -> Relational Operator/2
  Relational Operator/1 -> Enabled Subsystem/Enable
  Delay1/1 -> Subtract1/2
  dt/1 -> Enabled Subsystem/2(dt)
  Subtract1/1 -> Relational Operator/1
  Enabled Subsystem/1(dy/dt) -> dy/dt/1
  y/1 -> Enabled Subsystem/1(y), Delay1/1, Subtract1/1

== system Template_v5_0_0_2026a_Original/PhaseSpace Camera Code/Use Hardware to Obtain States/Store BLACK Data/Subsystem2 ==
  dt : Inport
  y : Inport  Port=2
  Constant3 : Constant  Value=0
  Delay1 : Delay  DelayLength=1
  Enabled Subsystem : Subsystem  TreatAsAtomicUnit=on
  Relational Operator : RelationalOperator  Operator=~=  OutDataTypeStr=boolean  RndMeth=Simplest  InputSameDT=off
  Subtract1 : Sum  Inputs=+-
  dy/dt : Outport
  wires:
  Constant3/1 -> Relational Operator/2
  Relational Operator/1 -> Enabled Subsystem/Enable
  Delay1/1 -> Subtract1/2
  dt/1 -> Enabled Subsystem/2(dt)
  Subtract1/1 -> Relational Operator/1
  Enabled Subsystem/1(dy/dt) -> dy/dt/1
  y/1 -> Enabled Subsystem/1(y), Delay1/1, Subtract1/1

== system Template_v5_0_0_2026a_Original/PhaseSpace Camera Code/Use Hardware to Obtain States/Store BLACK Data/Wrap ==
  Unwrapped Angle : Inport
  Atan2 : Trigonometry  Operator=atan2
  Cos : Trigonometry  Operator=cos
  Sin : Trigonometry
  Wrapped Angle : Outport
  wires:
  Unwrapped Angle/1 -> Sin/1, Cos/1
  Cos/1 -> Atan2/2
  Atan2/1 -> Wrapped Angle/1
  Sin/1 -> Atan2/1

== system Template_v5_0_0_2026a_Original/PhaseSpace Camera Code/Use Hardware to Obtain States/Store BLUE Data/Calculate True Time Step ==
  Time : Inport
  Data : Inport  Port=2
  Constant : Constant  Value=dataRate
  Constant3 : Constant  Value=0
  Delay1 : Delay  DelayLength=1  InitialCondition=0
  Delay2 : Delay  DelayLength=1  InitialCondition=0
  Demux : Demux  Outputs=3
  Enabled Subsystem3 : Subsystem  TreatAsAtomicUnit=on
  MATLAB Function : MATLAB Function  TreatAsAtomicUnit=on
  Relational Operator : RelationalOperator  Operator=~=  OutDataTypeStr=boolean  RndMeth=Simplest  InputSameDT=off
  Subtract1 : Sum  Inputs=+-
  Subtract2 : Sum  Inputs=+-
  Terminator : Terminator
  Terminator1 : Terminator
  dt_out : Outport
  wires:
  Demux/3 -> Terminator1/1
  Constant/1 -> MATLAB Function/2(dataRate)
  MATLAB Function/1(dt_out) -> dt_out/1
  Time/1 -> Delay2/1, Subtract1/1
  Enabled Subsystem3/1(dy(t)/dt) -> MATLAB Function/1(dt)
  Data/1 -> Demux/1
  Subtract2/1 -> Relational Operator/1
  Relational Operator/1 -> Enabled Subsystem3/Enable
  Constant3/1 -> Relational Operator/2
  Demux/1 -> Subtract2/1, Delay1/1
  Delay1/1 -> Subtract2/2
  Demux/2 -> Terminator/1
  Subtract1/1 -> Enabled Subsystem3/1(y2-y1)
  Delay2/1 -> Subtract1/2

== system Template_v5_0_0_2026a_Original/PhaseSpace Camera Code/Use Hardware to Obtain States/Store BLUE Data/Subsystem1 ==
  dt : Inport
  y : Inport  Port=2
  Constant3 : Constant  Value=0
  Delay1 : Delay  DelayLength=1
  Enabled Subsystem : Subsystem  TreatAsAtomicUnit=on
  Relational Operator : RelationalOperator  Operator=~=  OutDataTypeStr=boolean  RndMeth=Simplest  InputSameDT=off
  Subtract1 : Sum  Inputs=+-
  dy/dt : Outport
  wires:
  Constant3/1 -> Relational Operator/2
  Relational Operator/1 -> Enabled Subsystem/Enable
  Delay1/1 -> Subtract1/2
  dt/1 -> Enabled Subsystem/2(dt)
  Subtract1/1 -> Relational Operator/1
  Enabled Subsystem/1(dy/dt) -> dy/dt/1
  y/1 -> Enabled Subsystem/1(y), Delay1/1, Subtract1/1

== system Template_v5_0_0_2026a_Original/PhaseSpace Camera Code/Use Hardware to Obtain States/Store BLUE Data/Subsystem2 ==
  dt : Inport
  y : Inport  Port=2
  Constant3 : Constant  Value=0
  Delay1 : Delay  DelayLength=1
  Enabled Subsystem : Subsystem  TreatAsAtomicUnit=on
  Relational Operator : RelationalOperator  Operator=~=  OutDataTypeStr=boolean  RndMeth=Simplest  InputSameDT=off
  Subtract1 : Sum  Inputs=+-
  dy/dt : Outport
  wires:
  Constant3/1 -> Relational Operator/2
  Relational Operator/1 -> Enabled Subsystem/Enable
  Delay1/1 -> Subtract1/2
  dt/1 -> Enabled Subsystem/2(dt)
  Subtract1/1 -> Relational Operator/1
  Enabled Subsystem/1(dy/dt) -> dy/dt/1
  y/1 -> Enabled Subsystem/1(y), Delay1/1, Subtract1/1

== system Template_v5_0_0_2026a_Original/PhaseSpace Camera Code/Use Hardware to Obtain States/Store BLUE Data/Wrap ==
  Unwrapped Angle : Inport
  Atan2 : Trigonometry  Operator=atan2
  Cos : Trigonometry  Operator=cos
  Sin : Trigonometry
  Wrapped Angle : Outport
  wires:
  Unwrapped Angle/1 -> Sin/1, Cos/1
  Cos/1 -> Atan2/2
  Atan2/1 -> Wrapped Angle/1
  Sin/1 -> Atan2/1

== system Template_v5_0_0_2026a_Original/PhaseSpace Camera Code/Use Hardware to Obtain States/Store RED Data/Calculate True Time Step ==
  Time : Inport
  Data : Inport  Port=2
  Constant : Constant  Value=dataRate
  Constant3 : Constant  Value=0
  Delay1 : Delay  DelayLength=1  InitialCondition=0
  Delay2 : Delay  DelayLength=1  InitialCondition=0
  Demux : Demux  Outputs=3
  Enabled Subsystem3 : Subsystem  TreatAsAtomicUnit=on
  MATLAB Function : MATLAB Function  TreatAsAtomicUnit=on
  Relational Operator : RelationalOperator  Operator=~=  OutDataTypeStr=boolean  RndMeth=Simplest  InputSameDT=off
  Subtract1 : Sum  Inputs=+-
  Subtract2 : Sum  Inputs=+-
  Terminator : Terminator
  Terminator1 : Terminator
  dt_out : Outport
  wires:
  Demux/3 -> Terminator1/1
  Constant/1 -> MATLAB Function/2(dataRate)
  MATLAB Function/1(dt_out) -> dt_out/1
  Time/1 -> Delay2/1, Subtract1/1
  Enabled Subsystem3/1(dy(t)/dt) -> MATLAB Function/1(dt)
  Data/1 -> Demux/1
  Subtract2/1 -> Relational Operator/1
  Relational Operator/1 -> Enabled Subsystem3/Enable
  Constant3/1 -> Relational Operator/2
  Demux/1 -> Subtract2/1, Delay1/1
  Delay1/1 -> Subtract2/2
  Demux/2 -> Terminator/1
  Subtract1/1 -> Enabled Subsystem3/1(y2-y1)
  Delay2/1 -> Subtract1/2

== system Template_v5_0_0_2026a_Original/PhaseSpace Camera Code/Use Hardware to Obtain States/Store RED Data/Subsystem1 ==
  dt : Inport
  y : Inport  Port=2
  Constant3 : Constant  Value=0
  Delay1 : Delay  DelayLength=1
  Enabled Subsystem : Subsystem  TreatAsAtomicUnit=on
  Relational Operator : RelationalOperator  Operator=~=  OutDataTypeStr=boolean  RndMeth=Simplest  InputSameDT=off
  Subtract1 : Sum  Inputs=+-
  dy/dt : Outport
  wires:
  Constant3/1 -> Relational Operator/2
  Relational Operator/1 -> Enabled Subsystem/Enable
  Delay1/1 -> Subtract1/2
  dt/1 -> Enabled Subsystem/2(dt)
  Subtract1/1 -> Relational Operator/1
  Enabled Subsystem/1(dy/dt) -> dy/dt/1
  y/1 -> Enabled Subsystem/1(y), Delay1/1, Subtract1/1

== system Template_v5_0_0_2026a_Original/PhaseSpace Camera Code/Use Hardware to Obtain States/Store RED Data/Subsystem2 ==
  dt : Inport
  y : Inport  Port=2
  Constant3 : Constant  Value=0
  Delay1 : Delay  DelayLength=1
  Enabled Subsystem : Subsystem  TreatAsAtomicUnit=on
  Relational Operator : RelationalOperator  Operator=~=  OutDataTypeStr=boolean  RndMeth=Simplest  InputSameDT=off
  Subtract1 : Sum  Inputs=+-
  dy/dt : Outport
  wires:
  Constant3/1 -> Relational Operator/2
  Relational Operator/1 -> Enabled Subsystem/Enable
  Delay1/1 -> Subtract1/2
  dt/1 -> Enabled Subsystem/2(dt)
  Subtract1/1 -> Relational Operator/1
  Enabled Subsystem/1(dy/dt) -> dy/dt/1
  y/1 -> Enabled Subsystem/1(y), Delay1/1, Subtract1/1

== system Template_v5_0_0_2026a_Original/PhaseSpace Camera Code/Use Hardware to Obtain States/Store RED Data/Wrap ==
  Unwrapped Angle : Inport
  Atan2 : Trigonometry  Operator=atan2
  Cos : Trigonometry  Operator=cos
  Sin : Trigonometry
  Wrapped Angle : Outport
  wires:
  Unwrapped Angle/1 -> Sin/1, Cos/1
  Cos/1 -> Atan2/2
  Atan2/1 -> Wrapped Angle/1
  Sin/1 -> Atan2/1

== system Template_v5_0_0_2026a_Original/Simulate Plant Dynamics/BLACK Dynamics/Calculated & Store Measured States/Subsystem1 ==
  dt : Inport
  y : Inport  Port=2
  Constant3 : Constant  Value=0
  Delay1 : Delay  DelayLength=1
  Enabled Subsystem : Subsystem  TreatAsAtomicUnit=on
  Relational Operator : RelationalOperator  Operator=~=  OutDataTypeStr=boolean  RndMeth=Simplest  InputSameDT=off
  Subtract1 : Sum  Inputs=+-
  dy/dt : Outport
  wires:
  Constant3/1 -> Relational Operator/2
  Relational Operator/1 -> Enabled Subsystem/Enable
  Delay1/1 -> Subtract1/2
  dt/1 -> Enabled Subsystem/2(dt)
  Subtract1/1 -> Relational Operator/1
  Enabled Subsystem/1(dy/dt) -> dy/dt/1
  y/1 -> Enabled Subsystem/1(y), Delay1/1, Subtract1/1

== system Template_v5_0_0_2026a_Original/Simulate Plant Dynamics/BLACK Dynamics/Calculated & Store Measured States/Subsystem2 ==
  dt : Inport
  y : Inport  Port=2
  Constant3 : Constant  Value=0
  Delay1 : Delay  DelayLength=1
  Enabled Subsystem : Subsystem  TreatAsAtomicUnit=on
  Relational Operator : RelationalOperator  Operator=~=  OutDataTypeStr=boolean  RndMeth=Simplest  InputSameDT=off
  Subtract1 : Sum  Inputs=+-
  dy/dt : Outport
  wires:
  Constant3/1 -> Relational Operator/2
  Relational Operator/1 -> Enabled Subsystem/Enable
  Delay1/1 -> Subtract1/2
  dt/1 -> Enabled Subsystem/2(dt)
  Subtract1/1 -> Relational Operator/1
  Enabled Subsystem/1(dy/dt) -> dy/dt/1
  y/1 -> Enabled Subsystem/1(y), Delay1/1, Subtract1/1

== system Template_v5_0_0_2026a_Original/Simulate Plant Dynamics/BLACK Dynamics/Calculated & Store Measured States/Wrap ==
  Unwrapped Angle : Inport
  Atan2 : Trigonometry  Operator=atan2
  Cos : Trigonometry  Operator=cos
  Sin : Trigonometry
  Wrapped Angle : Outport
  wires:
  Unwrapped Angle/1 -> Sin/1, Cos/1
  Cos/1 -> Atan2/2
  Atan2/1 -> Wrapped Angle/1
  Sin/1 -> Atan2/1

== system Template_v5_0_0_2026a_Original/Simulate Plant Dynamics/BLACK Dynamics/Calculated & Store True States/Wrap ==
  Unwrapped Angle : Inport
  Atan2 : Trigonometry  Operator=atan2
  Cos : Trigonometry  Operator=cos
  Sin : Trigonometry
  Wrapped Angle : Outport
  wires:
  Unwrapped Angle/1 -> Sin/1, Cos/1
  Cos/1 -> Atan2/2
  Atan2/1 -> Wrapped Angle/1
  Sin/1 -> Atan2/1

== system Template_v5_0_0_2026a_Original/Simulate Plant Dynamics/BLACK Dynamics/Data @ Measurement Rate/Calculate True Time Step ==
  Data : Inport
  Time : Inport  Port=2
  Rate : Inport  Port=3
  Constant3 : Constant  Value=0
  Delay1 : Delay  DelayLength=1  InitialCondition=0
  Delay2 : Delay  DelayLength=1  InitialCondition=0
  Demux : Demux  Outputs=3
  Enabled Subsystem3 : Subsystem  TreatAsAtomicUnit=on
  MATLAB Function : MATLAB Function  TreatAsAtomicUnit=on
  Relational Operator : RelationalOperator  Operator=~=  OutDataTypeStr=boolean  RndMeth=Simplest  InputSameDT=off
  Subtract1 : Sum  Inputs=+-
  Subtract2 : Sum  Inputs=+-
  Terminator : Terminator
  Terminator1 : Terminator
  dt_out : Outport
  wires:
  Demux/3 -> Terminator1/1
  Rate/1 -> MATLAB Function/2(dataRate)
  MATLAB Function/1(dt_out) -> dt_out/1
  Time/1 -> Delay2/1, Subtract1/1
  Enabled Subsystem3/1(dy(t)/dt) -> MATLAB Function/1(dt)
  Data/1 -> Demux/1
  Subtract2/1 -> Relational Operator/1
  Relational Operator/1 -> Enabled Subsystem3/Enable
  Constant3/1 -> Relational Operator/2
  Demux/1 -> Subtract2/1, Delay1/1
  Delay1/1 -> Subtract2/2
  Demux/2 -> Terminator/1
  Subtract1/1 -> Enabled Subsystem3/1(y2-y1)
  Delay2/1 -> Subtract1/2

== system Template_v5_0_0_2026a_Original/Simulate Plant Dynamics/BLACK Dynamics/Data @ Measurement Rate/Enabled Subsystem ==
  In1 : Inport
  Enable : EnablePort
  Out1 : Outport
  wires:
  In1/1 -> Out1/1

== system Template_v5_0_0_2026a_Original/Simulate Plant Dynamics/BLACK Dynamics/Data @ Measurement Rate/Enabled Subsystem1 ==
  ThrustPer_Final : Inport
  Enable : EnablePort
  Out1 : Outport
  wires:
  ThrustPer_Final/1 -> Out1/1
